simulink model "MATLAB_Arduino_ICM20689_Real_Time"  (R2021a)
settings: Solver=FixedStepAuto  StartTime=0.0  StopTime=10  RelTol=1e-3  EnableMultiTasking=on
libraries: arduinolib x5, sldrtlib x1
settings Model: SILPILModeSetting=veronly  ExtModeTrigDuration=2  Creator=mpnoy  LastModifiedBy=mpnoy
settings OptimizationCC: EnhancedBackFolding=on  PassReuseOutputArgsAs=Individual arguments  ZeroExternalMemoryAtStartup=off  ZeroInternalMemoryAtStartup=off  MaxStackSize=64  OptimizeBlockOrder=speed  DifferentSizesBufferReuse=on  OptimizationCustomize=off  EfficientTunableParamExpr=on
settings DebuggingCC: ParameterTunabilityLossMsg=error
settings HardwareCC: ProdBitPerInt=16  ProdBitPerPointer=16  ProdBitPerSizeT=16  ProdBitPerPtrDiffT=16  ProdLargestAtomicFloat=None  ProdWordSize=8  ProdHWDeviceType=Atmel->AVR
settings SFSimCC: MATLABDynamicMemAlloc=off
settings RTWCC: SystemTargetFile=ert.tlc  HardwareBoard=Arduino Uno  TemplateMakefile=ert_default_tmf  Toolchain=Arduino AVR  BuildConfiguration=Faster Runs
settings CodeAppCC: ForceParamTrailComments=on  IgnoreCustomStorageClasses=off  OperatorAnnotations=on  SimulinkDataObjDesc=on  SFDataObjDesc=on  InsertBlockDesc=on
settings ERTTargetCC: SupportContinuousTime=on  SupportVariableSizeSignals=on  ExtModeStaticAllocSize=250

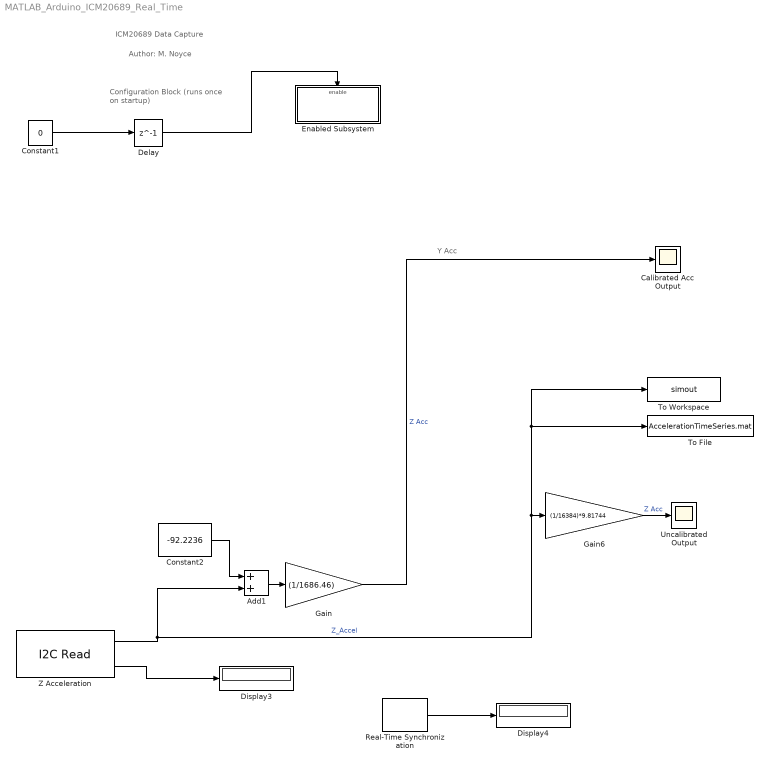
== system MATLAB_Arduino_ICM20689_Real_Time ==
  note: Y Acc
  note: Author: M. Noyce
  note: ICM20689 Data Capture
  note: Configuration Block
      | (runs once on startup)
  Add1 : Sum
  "Calibrated Acc Output " : Scope
  Constant1 : Constant  Value=0
  Constant2 : Constant  Value=-92.2236
  Delay : Delay  DelayLength=1  InitialCondition=1
  Display3 : Display
  Display4 : Display
  Enabled Subsystem : Subsystem  TreatAsAtomicUnit=on
  Gain : Gain  Gain=(1/1686.46)
  Gain6 : Gain  Gain=(1/16384)*9.81744
  Real-Time Synchronization : sldrtlib/Real-Time Synchronization  SampleTime=0.1  MaxMissedTicks=10  ShowMissedTicks=on  YieldWhenWaiting=on
  To File : ToFile  Filename=AccelerationTimeSeries.mat  MatrixName=Acceleration  SaveFormat=Timeseries
  To Workspace : ToWorkspace  VariableName=simout  SaveFormat=Timeseries  SampleTime=-1
  "Uncalibrated Output " : Scope
  "Z Acceleration " : arduinolib/I2C Read  I2CModule=0  Mode=Master  SlaveAddress=104  SlaveByteOrder=BigEndian  Direction=Receiver  RegisterAddressMode=on  RegisterAddress=uint8(hex2dec('3F'))  SlaveDataType=int16  DataLength=1  NoAck=off  RepeatedStart=off  OutputStatus=on  blockPlatform=ARDUINO  SampleTime=0.01
      settings: SourceProductBaseCode=ARDUINO
  wires:
  Constant1/1 -> Delay/1
  Delay/1 -> Enabled Subsystem/Enable
  "Z Acceleration "/2 -> Display3/1
  "Z Acceleration "/1 -> To Workspace/1, To File/1, Gain6/1, Add1/2  "Z_Accel"
  Constant2/1 -> Add1/1
  Gain/1 -> "Calibrated Acc Output "/1  "Z Acc"
  Add1/1 -> Gain/1
  Gain6/1 -> "Uncalibrated Output "/1  "Z Acc"
  Real-Time Synchronization/1 -> Display4/1

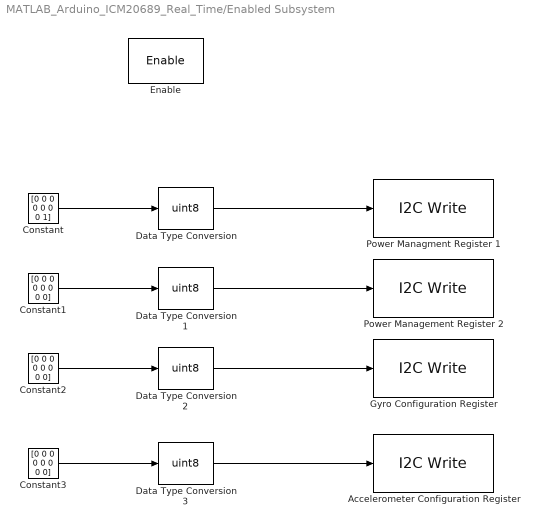
== system MATLAB_Arduino_ICM20689_Real_Time/Enabled Subsystem ==
  Enable : EnablePort
  "Accelerometer Configuration Register " : arduinolib/I2C Write  I2CModule=0  Mode=Master  SlaveAddress=104  SlaveByteOrder=BigEndian  Direction=Transmitter  RegisterAddressMode=on  RegisterAddress=uint8(hex2dec('1C'))  SlaveDataType=uint8  DataLength=1  NoAck=off  RepeatedStart=off  OutputStatus=off  blockPlatform=ARDUINO
      settings: SourceProductBaseCode=ARDUINO
  Constant : Constant  Value=[0 0 0 0 0 0 0 1]
  Constant1 : Constant  Value=[0 0 0 0 0 0 0 0]
  Constant2 : Constant  Value=[0 0 0 0 0 0 0 0]
  Constant3 : Constant  Value=[0 0 0 0 0 0 0 0]
  Data Type Conversion{,1..3} (4 alike) : DataTypeConversion  OutDataTypeStr=uint8
  Gyro Configuration Register : arduinolib/I2C Write  I2CModule=0  Mode=Master  SlaveAddress=104  SlaveByteOrder=BigEndian  Direction=Transmitter  RegisterAddressMode=on  RegisterAddress=uint8(hex2dec('1B'))  SlaveDataType=uint8  DataLength=1  NoAck=off  RepeatedStart=off  OutputStatus=off  blockPlatform=ARDUINO
      settings: SourceProductBaseCode=ARDUINO
  Power Management Register 2 : arduinolib/I2C Write  I2CModule=0  Mode=Master  SlaveAddress=104  SlaveByteOrder=BigEndian  Direction=Transmitter  RegisterAddressMode=on  RegisterAddress=uint8(hex2dec('6C'))  SlaveDataType=uint8  DataLength=1  NoAck=off  RepeatedStart=off  OutputStatus=off  blockPlatform=ARDUINO
      settings: SourceProductBaseCode=ARDUINO
  "Power Managment Register 1 " : arduinolib/I2C Write  I2CModule=0  Mode=Master  SlaveAddress=104  SlaveByteOrder=BigEndian  Direction=Transmitter  RegisterAddressMode=on  RegisterAddress=uint8(hex2dec('6B'))  SlaveDataType=uint8  DataLength=1  NoAck=off  RepeatedStart=off  OutputStatus=off  blockPlatform=ARDUINO
      settings: SourceProductBaseCode=ARDUINO
  wires:
  Data Type Conversion/1 -> "Power Managment Register 1 "/1
  Constant/1 -> Data Type Conversion/1
  Constant1/1 -> Data Type Conversion1/1
  Data Type Conversion1/1 -> Power Management Register 2/1
  Data Type Conversion2/1 -> Gyro Configuration Register/1
  Constant2/1 -> Data Type Conversion2/1
  Data Type Conversion3/1 -> "Accelerometer Configuration Register "/1
  Constant3/1 -> Data Type Conversion3/1
